simulink library "sf_msg_traffic_light_lib"  (R2025b)
settings: Solver=ode45  StartTime=0.0  StopTime=10.0  RelTol=1e-3  EnableMultiTasking=on
settings Model: Creator=The MathWorks, Inc.  LastModifiedBy=The MathWorks, Inc.
settings SolverCC: AlgebraicLoopSolver=TrustRegion
settings DataIOCC: LimitDataPoints=on  SaveFormat=Array  ReturnWorkspaceOutputs=off
settings OptimizationCC: ReuseModelBlockBuffer=off  LifeSpan=inf
settings DebuggingCC: SolverPrmCheckMsg=warning  UnconnectedInputMsg=warning  UnconnectedOutputMsg=warning  UnconnectedLineMsg=warning  AllowSymbolicDim=off  PregeneratedLibrarySubsystemCodeDiagnostic=none  SFUnexpectedBacktrackingDiag=warning  SFNoUnconditionalDefaultTransitionDiag=warning  SFExecutionAtInitializationDiag=none  ArithmeticOperatorsInVariantConditions=warning
settings HardwareCC: ProdBitPerPointer=32.0  ProdBitPerSizeT=32.0  ProdBitPerPtrDiffT=32.0  ProdLargestAtomicFloat=None  ProdIntDivRoundTo=Undefined  ProdEndianess=Unspecified  ProdWordSize=32.0  ProdHWDeviceType=32-bit Generic
settings ModelReferenceCC: EnableRefExpFcnMdlSchedulingChecks=on  PropagateSignalLabelsOutOfModel=off
settings SFSimCC: SimUseLocalCustomCode=off  CustomCodeUndefinedFunction=UseInterfaceOnly
settings RTWCC: RTWUseLocalCustomCode=off  GPUComputeCapability=3.5
settings CodeAppCC: StateflowObjectComments=on
settings GRTTargetCC: TargetLangStandard=C89/C90 (ANSI)
settings ConfigComp: CovMetricSettings=dw  CovSaveCumulativeToWorkspaceVar=on  CovSaveSingleToWorkspaceVar=on  CovExternalEMLEnable=off  CovSFcnEnable=off

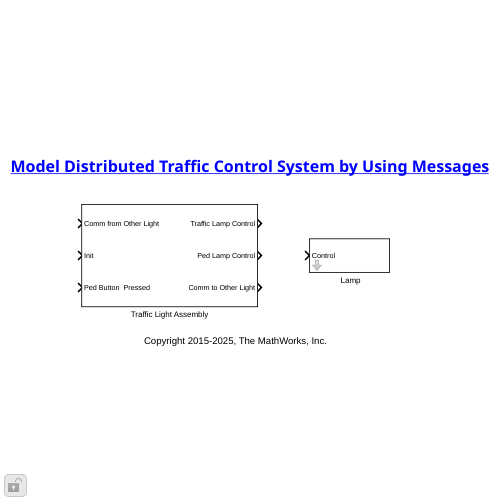
[thumbnail: Simulink's stored preview of the top-level diagram]
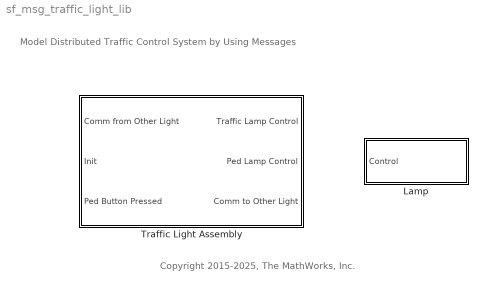
== system sf_msg_traffic_light_lib ==
  note: Copyright 2015-2025, The MathWorks, Inc.
  note: Model Distributed Traffic Control System by Using Messages
  " Lamp" : Subsystem  mask{LampSelect=Traffic Lamp 1}
      mask prompts: LampSelect "Lamp Select"
      mask TypeOptions LampSelect: Traffic Lamp 1 | Traffic Lamp 2 | Ped Lamp 1 | Ped Lamp 2
  Traffic Light Assembly : Subsystem

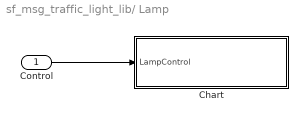
== system sf_msg_traffic_light_lib/ Lamp ==
  Control : Inport
  Chart : Stateflow chart  TreatAsAtomicUnit=on
  wires:
  Control/1 -> Chart/1(LampControl)

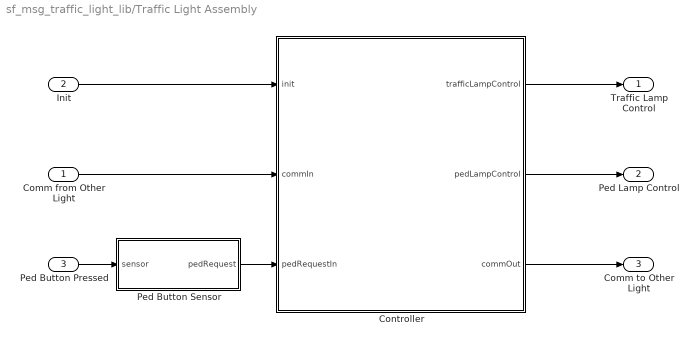
== system sf_msg_traffic_light_lib/Traffic Light Assembly ==
  Comm from Other Light : Inport
  Init : Inport  Port=2
  Ped Button Pressed : Inport  Port=3
  Controller : Stateflow chart  TreatAsAtomicUnit=on
      settings: RTWSystemCode=Reusable function
  Ped Button Sensor : Stateflow chart  TreatAsAtomicUnit=on
      settings: RTWSystemCode=Inline
  Traffic Lamp Control : Outport  VectorParamsAs1DForOutWhenUnconnected=off
  Ped Lamp Control : Outport  Port=2  VectorParamsAs1DForOutWhenUnconnected=off
  Comm to Other Light : Outport  Port=3  VectorParamsAs1DForOutWhenUnconnected=off
  wires:
  Ped Button Pressed/1 -> Ped Button Sensor/1(sensor)
  Controller/2(pedLampControl) -> Ped Lamp Control/1
  Controller/1(trafficLampControl) -> Traffic Lamp Control/1
  Comm from Other Light/1 -> Controller/2(commIn)
  Controller/3(commOut) -> Comm to Other Light/1
  Init/1 -> Controller/1(init)
  Ped Button Sensor/1(pedRequest) -> Controller/3(pedRequestIn)

== stateflow chart sf_msg_traffic_light_lib/Traffic Light Assembly/Controller ==
  state PedCrossing
    en:
    pedLampControl.data = GREEN;
    send(pedLampControl);
  state NormalCycle
    en:
    pedLampControl.data = RED;
    send(pedLampControl);
    (history)
    state Stop
      en:
      commOut.data = STOPPED;
      send(commOut);
      on pedRequestIn:
      forward(pedRequestIn,commOut);
      on pedRequestLocal:
      forward(pedRequestLocal,commOut);
    state PrepareToGo
      en:
      commOut.data = REQ_STOP;
      send(commOut);
    state PrepareToStop
    state Go
    (default) -> Stop [order 1] : [init == 0]
    (junction 114) -> (junction 76) [order 1] : [readyForPed]
    (junction 114) -> Stop [order 2]
    Stop -> PrepareToGo : after(3,sec)
        | {readyForPed = true;}
    PrepareToStop -> (junction 114) : after(1,sec)
        | {
        | trafficLampControl.data = RED;
        | send(trafficLampControl);
        | }
    PrepareToGo -> (junction 95) : commIn
        | [commIn.data == STOPPED]
    (default) -> (junction 95) [order 2]
    (junction 95) -> Go : {
        | trafficLampControl.data = GREEN;
        | send(trafficLampControl);
        | }
    (junction 97) -> PrepareToStop [order 1] : [commIn.data == REQ_STOP]
        | {
        | trafficLampControl.data = YELLOW;
        | send(trafficLampControl);
        | }
    (junction 97) -> Go [order 2] : [commIn.data == REQ_PED]
        | /{forward(commIn,pedRequestLocal);}
    (junction 121) -> (junction 97)
    Go -> (junction 123)
    (junction 123) -> (junction 121) : commIn
  (junction 112) -> PedCrossing : {commOut.data = PED;
      | send(commOut);}
  NormalCycle -> PedCrossing : commIn
      | [commIn.data == PED]
  (junction 76) -> (junction 112) [order 1] : pedRequestIn
  (junction 76) -> (junction 112) [order 2] : pedRequestLocal
  PedCrossing -> NormalCycle : after(3,sec)
      | {readyForPed = false;}
  (default) -> NormalCycle
  data: init input size=1; commIn input Enum: trafficComms size=1; pedRequestIn input Enum: trafficComms; trafficLampControl output Enum: trafficColors size=1; pedLampControl output Enum: trafficColors size=1; commOut output Enum: trafficComms size=1; pedRequestLocal local Enum: trafficComms size=1; readyForPed local =true

== stateflow chart sf_msg_traffic_light_lib/ Lamp/Chart ==
  state Wait
  state Set
    en:
    changeLamp(LampControl.data);
  (default) -> Wait
  Set -> Wait
  Wait -> Set : LampControl
  data: next function_input; LampSelect parameter size=1; LampControl input Enum: trafficColors size=1
  function changeLamp(next):
    | function changeLamp(next)
    |     coder.extrinsic('tl_gui');
    |     switch LampSelect
    |         case 3 % 'Ped Lamp 1'
    |             tl_gui('onp',1,next);
    |         case 4 % 'Ped Lamp 2'
    |             tl_gui('onp',2,next);
    |         case 1 % 'Traffic Lamp 1'
    |             tl_gui('ont',1,next);
    |         case 2 % 'Traffic Lamp 2'
    |             tl_gui('ont',2,next);
    |     end
    | end

== stateflow chart sf_msg_traffic_light_lib/Traffic Light Assembly/Ped Button Sensor ==
  state sensing
  (default) -> sensing : {currValue=sensor;}
  sensing -> sensing : [sensor~=currValue]
      | /{
      | currValue=sensor;
      | pedRequest.data=REQ_PED;
      | send(pedRequest);
      | }
  data: sensor input; currValue local double size=1; pedRequest output Enum: trafficComms size=1
